simulink model "hamming_dec"  (R2023b)
settings: Solver=FixedStepDiscrete  StartTime=0.0  StopTime=463  FixedStep=1  RelTol=1e-3
libraries: simulink x5
settings Model: Creator=e2507457  LastModifiedBy=e2507457

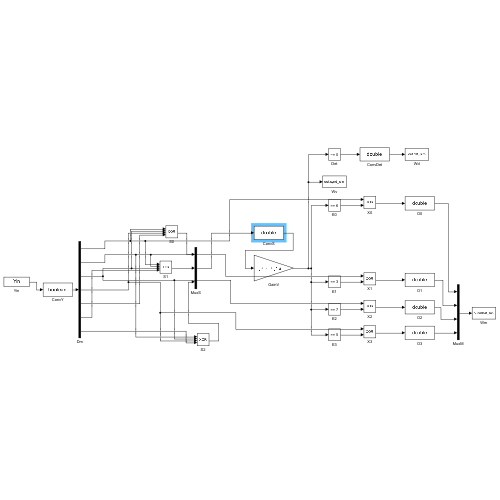
[thumbnail: Simulink's stored preview of the top-level diagram]
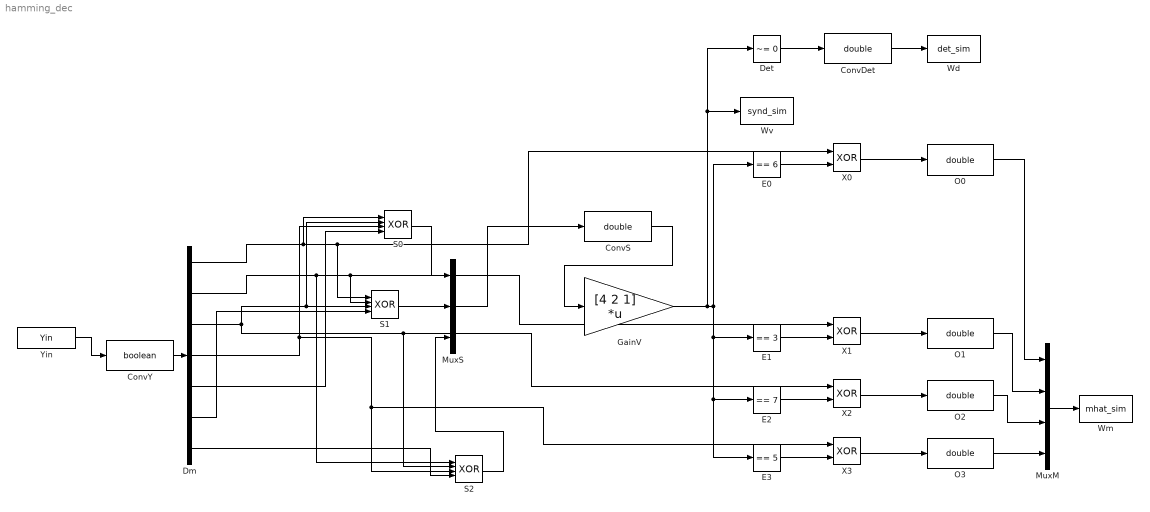
== system hamming_dec ==
  ConvDet : DataTypeConversion  OutDataTypeStr=double  SaturateOnIntegerOverflow=off  RndMeth=Floor
  ConvS : DataTypeConversion  OutDataTypeStr=double  SaturateOnIntegerOverflow=off  RndMeth=Floor
  ConvY : DataTypeConversion  OutDataTypeStr=boolean  SaturateOnIntegerOverflow=off  RndMeth=Floor
  Det : simulink/Logic and Bit Operations/Compare To Constant  relop=~=  const=0  OutDataTypeStr=boolean
  Dm : Demux  Outputs=7
  E0 : simulink/Logic and Bit Operations/Compare To Constant  relop===  const=6  OutDataTypeStr=boolean
  E1 : simulink/Logic and Bit Operations/Compare To Constant  relop===  const=3  OutDataTypeStr=boolean
  E2 : simulink/Logic and Bit Operations/Compare To Constant  relop===  const=7  OutDataTypeStr=boolean
  E3 : simulink/Logic and Bit Operations/Compare To Constant  relop===  const=5  OutDataTypeStr=boolean
  GainV : Gain  Gain=[4 2 1]  Multiplication=Matrix(K*u)
  MuxM : Mux
  MuxS : Mux  Inputs=3
  O{0..3} (4 alike) : DataTypeConversion  OutDataTypeStr=double  SaturateOnIntegerOverflow=off  RndMeth=Floor
  S0 : Logic  Operator=XOR  Inputs=4  AllPortsSameDT=off  OutDataTypeStr=boolean
  S1 : Logic  Operator=XOR  Inputs=4  AllPortsSameDT=off  OutDataTypeStr=boolean
  S2 : Logic  Operator=XOR  Inputs=4  AllPortsSameDT=off  OutDataTypeStr=boolean
  Wd : ToWorkspace  VariableName=det_sim  SampleTime=-1
  Wm : ToWorkspace  VariableName=mhat_sim  SampleTime=-1
  Wv : ToWorkspace  VariableName=synd_sim  SampleTime=-1
  X{0..3} (4 alike) : Logic  Operator=XOR  AllPortsSameDT=off  OutDataTypeStr=boolean
  Yin : FromWorkspace  VariableName=Yin  SampleTime=1  Interpolate=off  OutputAfterFinalValue=Holding final value
  wires:
  O0/1 -> MuxM/1
  ConvY/1 -> Dm/1
  Yin/1 -> ConvY/1
  Dm/1 -> X0/1, S1/1, S0/1
  Dm/2 -> X1/1, S1/2, S2/1
  Dm/3 -> S0/2, S1/3, S2/2, X2/1
  Dm/4 -> S0/3, S2/3, X3/1
  Dm/5 -> S0/4
  Dm/6 -> S1/4
  MuxS/1 -> ConvS/1
  Dm/7 -> S2/4
  S0/1 -> MuxS/1
  S1/1 -> MuxS/2
  O3/1 -> MuxM/4
  S2/1 -> MuxS/3
  ConvS/1 -> GainV/1
  GainV/1 -> E2/1, E3/1, E1/1, E0/1, Det/1, Wv/1
  Det/1 -> ConvDet/1
  X0/1 -> O0/1
  E0/1 -> X0/2
  X1/1 -> O1/1
  E1/1 -> X1/2
  E2/1 -> X2/2
  E3/1 -> X3/2
  ConvDet/1 -> Wd/1
  X2/1 -> O2/1
  X3/1 -> O3/1
  O1/1 -> MuxM/2
  O2/1 -> MuxM/3
  MuxM/1 -> Wm/1
